simulink model "ECU1119_18b_st"  (R2018b)
settings: Solver=FixedStepDiscrete  StartTime=0.0  StopTime=10.0  RelTol=1e-3
InitFcn:
  | mbd_mpc_consistency_checks(bdroot(gcs));
values from neighbouring files (symbols this model uses):
  ANRtarget = 1.05    [Engine_init.m]
  EGRKi = 0.03    [Engine_init.m]
  EGRKp = 1.2*3    (= 3.6)    [Engine_init.m]
  EGRMax = 1    [Engine_init.m]
  EGRMin = 0    [Engine_init.m]
  EGRTgt = [0.25,0.22,0.20,0.18,0.16,0.12,0.10 ... (first row only)    [Engine_init.m]
  EGRTgt_x = [700,1200,1400,1600,1800,2000,2200]    [Engine_init.m]
  EGRTgt_y = [20,60,100,140,160]    [Engine_init.m]
  EngineSpdTgt = [700:150:2200]    [Engine_init.m]
  EngineSpdTgt_x = [0:10:100]    [Engine_init.m]
  FuelCyleMax = [40,50,60,60,60 ... (first row only)    [Engine_init.m]
  FuelCyleMax_x = [120,180,240,300,360]    [Engine_init.m]
  FuelCyleMax_y = [700,1200,1400,1600,1800,2000,2200]    [Engine_init.m]
  FuelCyleMaxSw = 0    [Engine_init.m]
  FuelCyleMin = 10    [Engine_init.m]
  FuelKd = 0    [Engine_init.m]
  FuelKi = 0.009*5    (= 0.045)    [Engine_init.m]
  FuelKp = 0.03*5    (= 0.15)    [Engine_init.m]
  Regen_Enable_SW = true    [Engine_init.m]
  Soot_Load_Off = 4    [Engine_init.m]
  Soot_Load_On = 18    [Engine_init.m]
  T_regen_max = 680    [Engine_init.m]
  T_regen_min = 550    [Engine_init.m]
undefined symbols (not defined in the file or in its folder): fifo_0_vect, fifo_1_vect, LQFP, pts1_fifo_0_vect, pts1_fifo_1_vect, pts2_fifo_0_vect, pts2_fifo_1_vect, pts3_fifo_0_vect, pts3_fifo_1_vect, pts4_fifo_0_vect, pts4_fifo_1_vect
libraries: mbd_mpc574x_ec_toolbox x111, simulink x12, canmsglib x8
(part 3 of 5)

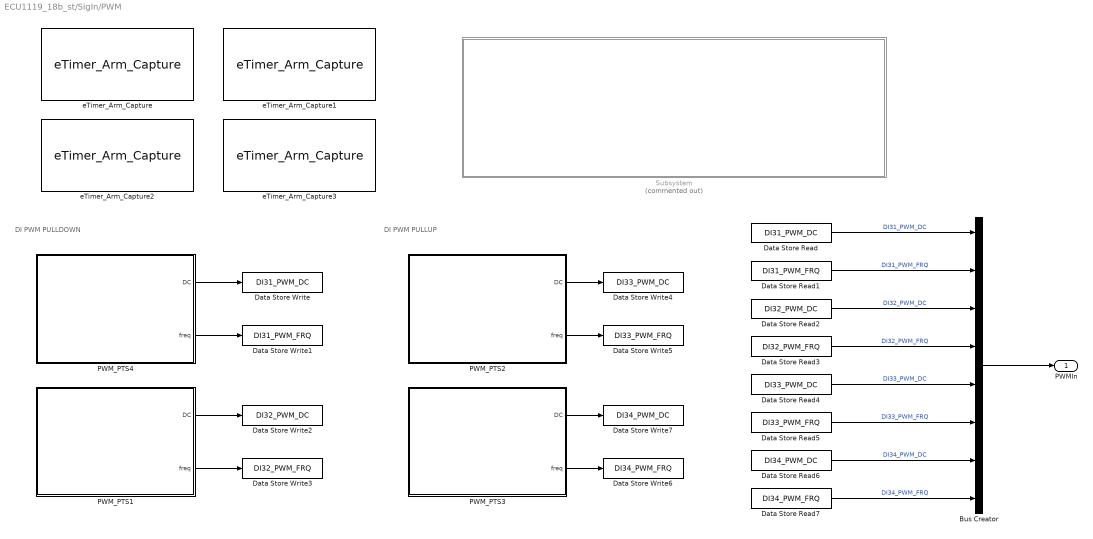
== system ECU1119_18b_st/SigIn/PWM ==
  note: DI PWM PULLDOWN
  note: DI PWM PULLUP
  Bus Creator : BusCreator  Inputs=8
  Data Store Read : DataStoreRead  DataStoreName=DI31_PWM_DC
  Data Store Read1 : DataStoreRead  DataStoreName=DI31_PWM_FRQ
  Data Store Read2 : DataStoreRead  DataStoreName=DI32_PWM_DC
  Data Store Read3 : DataStoreRead  DataStoreName=DI32_PWM_FRQ
  Data Store Read4 : DataStoreRead  DataStoreName=DI33_PWM_DC
  Data Store Read5 : DataStoreRead  DataStoreName=DI33_PWM_FRQ
  Data Store Read6 : DataStoreRead  DataStoreName=DI34_PWM_DC
  Data Store Read7 : DataStoreRead  DataStoreName=DI34_PWM_FRQ
  Data Store Write : DataStoreWrite  DataStoreName=DI31_PWM_DC
  Data Store Write1 : DataStoreWrite  DataStoreName=DI31_PWM_FRQ
  Data Store Write2 : DataStoreWrite  DataStoreName=DI32_PWM_DC
  Data Store Write3 : DataStoreWrite  DataStoreName=DI32_PWM_FRQ
  Data Store Write4 : DataStoreWrite  DataStoreName=DI33_PWM_DC
  Data Store Write5 : DataStoreWrite  DataStoreName=DI33_PWM_FRQ
  Data Store Write6 : DataStoreWrite  DataStoreName=DI34_PWM_FRQ
  Data Store Write7 : DataStoreWrite  DataStoreName=DI34_PWM_DC
  PWM_PTS1 : Subsystem
  PWM_PTS2 : Subsystem
  PWM_PTS3 : Subsystem
  PWM_PTS4 : Subsystem
  Subsystem : Subsystem  Commented=on
  eTimer_Arm_Capture : mbd_mpc574x_ec_toolbox/Motor Control Blocks/eTIMER Blocks/eTimer_Arm_Capture  etimerModule=0  etimerChannel=2  etimerArmAction=Start
      settings: SourceProductName=NXP Model-Based Design Toolbox for MPC57xx MCUs
  eTimer_Arm_Capture1 : mbd_mpc574x_ec_toolbox/Motor Control Blocks/eTIMER Blocks/eTimer_Arm_Capture  etimerModule=1  etimerChannel=2  etimerArmAction=Start
      settings: SourceProductName=NXP Model-Based Design Toolbox for MPC57xx MCUs
  eTimer_Arm_Capture2 : mbd_mpc574x_ec_toolbox/Motor Control Blocks/eTIMER Blocks/eTimer_Arm_Capture  etimerModule=1  etimerChannel=1  etimerArmAction=Start
      settings: SourceProductName=NXP Model-Based Design Toolbox for MPC57xx MCUs
  eTimer_Arm_Capture3 : mbd_mpc574x_ec_toolbox/Motor Control Blocks/eTIMER Blocks/eTimer_Arm_Capture  etimerModule=1  etimerChannel=3  etimerArmAction=Start
      settings: SourceProductName=NXP Model-Based Design Toolbox for MPC57xx MCUs
  PWMIn : Outport
  wires:
  Bus Creator/1 -> PWMIn/1
  Data Store Read7/1 -> Bus Creator/8  "DI34_PWM_FRQ"
  Data Store Read6/1 -> Bus Creator/7  "DI34_PWM_DC"
  Data Store Read5/1 -> Bus Creator/6  "DI33_PWM_FRQ"
  Data Store Read4/1 -> Bus Creator/5  "DI33_PWM_DC"
  Data Store Read3/1 -> Bus Creator/4  "DI32_PWM_FRQ"
  Data Store Read2/1 -> Bus Creator/3  "DI32_PWM_DC"
  Data Store Read1/1 -> Bus Creator/2  "DI31_PWM_FRQ"
  Data Store Read/1 -> Bus Creator/1  "DI31_PWM_DC"
  PWM_PTS4/1(DC) -> Data Store Write/1
  PWM_PTS4/2(freq) -> Data Store Write1/1
  PWM_PTS1/1(DC) -> Data Store Write2/1
  PWM_PTS1/2(freq) -> Data Store Write3/1
  PWM_PTS2/1(DC) -> Data Store Write4/1
  PWM_PTS2/2(freq) -> Data Store Write5/1
  PWM_PTS3/2(freq) -> Data Store Write6/1
  PWM_PTS3/1(DC) -> Data Store Write7/1

== system ECU1119_18b_st/SigOut/VCU_Cmd_Fast ==
  "EngCmd " : Inport
  Trigger : TriggerPort  VariantControl=Variant  PortDimensions=1
  Add : Sum
  Bus Selector : BusSelector  OutputSignals=Data,Length
  Bus Selector1 : BusSelector  OutputSignals=DPF_regen_req,EGROpeningTgt_pct,EngineSpdTgt_rpm,FuelCyleTgt_mg,PostInj_Request
  Constant2 : Constant  OutDataTypeStr=uint8
  Data Store Read : DataStoreRead  DataStoreName=Cnt_FAST_OUT
  Data Store Write : DataStoreWrite  DataStoreName=Cnt_FAST_OUT
  Data Type Conversion{,1..4} (5 alike) : DataTypeConversion  OutDataTypeStr=double
  FCAN_Send_ID_0x18FF0800 : mbd_mpc574x_ec_toolbox/Communication Blocks/CAN Blocks/FCAN_Send  Priority=2  can_instance=2  can_mode=Non-blocking  can_timeout_ms=0  can_mb_idx=6  can_extended_id=off  can_is_remote=off  can_id=107  show_adv_opts=off  can_fd_enable=off  can_enable_brs=off  can_fd_padding=0
      settings: SourceProductName=NXP Model-Based Design Toolbox for MPC57xx MCUs
  VCU_Cmd_Fast : canmsglib/CAN Pack  CANdbFile=D:\VCU\VCU_Tractor_HaerBin\Tractor2\CANtest\ECU_CAN_st.dbc  MsgList=VCU_Cmd_Fast  MsgName=VCU_Cmd_Fast  MsgIDType=Standard (11-bit identifier)  MsgIdentifier=263  MsgLength=8  SignalInfo=DPF_regen_req$56$8$1$2$1$0$1$0$0$1$#EGROpeningTgt_pct$32$16$1$2$1$0$1.000000e-02$0$0$100$#EngSpdTgt_rpm$0$16$1$2$1$0$1.000000e-01$0$0$3000$#FuelCycleTgt_mg$16$16$1$2$1$0$5.000000e-03$0$0$200$#PostInj_Request$48$8$1$2$1$0$1$0$0$1$#  NSignals=5  StartBits=str2num('[int32(56);int32(32);int32(0);int32(16);int32(48)]')  SignalSizes=str2num('[int32(8);int32(16);int32(16);int32(16);int32(8)]')  ByteOrders=str2num('[int32(1);int32(1);int32(1);int32(1);int32(1)]')  DataTypes=str2num('[int32(2);int32(2);int32(2);int32(2);int32(2)]')  MultiplexTypes=str2num('[int32(1);int32(1);int32(1);int32(1);int32(1)]')  MultiplexValues=str2num('[double(0);double(0);double(0);double(0);double(0)]')  Factors=str2num('[double(1);double(1.000000e-02);double(1.000000e-01);double(5.000000e-03);double(1)]')  Offsets=str2num('[double(0);double(0);double(0);double(0);double(0)]')  Minimums=str2num('[double(0);double(0);double(0);double(0);double(0)]')  Maximums=str2num('[double(1);double(100);double(3000);double(200);double(1)]')  Remote=off  ApplyMinMax=off  BusOutput=on
      settings: SourceProductName=Simulink Real-Time  SourceProductBaseCode=XP  DataFormat=CANdb specified signals
  wires:
  VCU_Cmd_Fast/1 -> Bus Selector/1
  Bus Selector/2 -> FCAN_Send_ID_0x18FF0800/2  "<Length>"
  Bus Selector/1 -> FCAN_Send_ID_0x18FF0800/1  "<Data>"
  Add/1 -> Data Store Write/1
  Data Store Read/1 -> Add/1
  Constant2/1 -> Add/2
  "EngCmd "/1 -> Bus Selector1/1
  Data Type Conversion/1 -> VCU_Cmd_Fast/1
  Data Type Conversion4/1 -> VCU_Cmd_Fast/5
  Data Type Conversion3/1 -> VCU_Cmd_Fast/4
  Data Type Conversion2/1 -> VCU_Cmd_Fast/3
  Data Type Conversion1/1 -> VCU_Cmd_Fast/2
  Bus Selector1/5 -> Data Type Conversion4/1  "<PostInj_Request>"
  Bus Selector1/4 -> Data Type Conversion3/1  "<FuelCyleTgt_mg>"
  Bus Selector1/3 -> Data Type Conversion2/1  "<EngineSpdTgt_rpm>"
  Bus Selector1/2 -> Data Type Conversion1/1  "<EGROpeningTgt_pct>"
  Bus Selector1/1 -> Data Type Conversion/1  "<DPF_regen_req>"

== system ECU1119_18b_st/SigOut/VCU_Cmd_Slow ==
  "EngCmd " : Inport
  Trigger : TriggerPort  VariantControl=Variant  PortDimensions=1
  Add : Sum
  Bus Selector : BusSelector  OutputSignals=Data,Length
  Bus Selector1 : BusSelector  OutputSignals=mUREA_target
  Constant : Constant  Value=0  OutDataTypeStr=single
  Constant2 : Constant  OutDataTypeStr=uint8
  Data Store Read : DataStoreRead  DataStoreName=Cnt_SLOW_OUT
  Data Store Write : DataStoreWrite  DataStoreName=Cnt_SLOW_OUT
  Data Type Conversion : DataTypeConversion  OutDataTypeStr=double
  Data Type Conversion1 : DataTypeConversion  OutDataTypeStr=double
  FCAN_Send_ID_0x18FF0900 : mbd_mpc574x_ec_toolbox/Communication Blocks/CAN Blocks/FCAN_Send  Priority=2  can_instance=2  can_mode=Non-blocking  can_timeout_ms=0  can_mb_idx=7  can_extended_id=off  can_is_remote=off  can_id=108  show_adv_opts=off  can_fd_enable=off  can_enable_brs=off  can_fd_padding=0
      settings: SourceProductName=NXP Model-Based Design Toolbox for MPC57xx MCUs
  VCU_Cmd_Slow : canmsglib/CAN Pack  CANdbFile=D:\VCU\VCU_Tractor_HaerBin\Tractor2\CANtest\ECU_CAN_st.dbc  MsgList=VCU_Cmd_Slow  MsgName=VCU_Cmd_Slow  MsgIDType=Standard (11-bit identifier)  MsgIdentifier=264  MsgLength=8  SignalInfo=Reserved_0900$0$32$1$3$1$0$1$0$-3.400000e+38$3.400000e+38$#mUREA_target_gph$32$32$1$3$1$0$1.000000e-01$0$-3.400000e+37$3.400000e+37$#  NSignals=2  StartBits=str2num('[int32(0);int32(32)]')  SignalSizes=str2num('[int32(32);int32(32)]')  ByteOrders=str2num('[int32(1);int32(1)]')  DataTypes=str2num('[int32(3);int32(3)]')  MultiplexTypes=str2num('[int32(1);int32(1)]')  MultiplexValues=str2num('[double(0);double(0)]')  Factors=str2num('[double(1);double(1.000000e-01)]')  Offsets=str2num('[double(0);double(0)]')  Minimums=str2num('[double(-3.400000e+38);double(-3.400000e+37)]')  Maximums=str2num('[double(3.400000e+38);double(3.400000e+37)]')  Remote=off  ApplyMinMax=off  BusOutput=on
      settings: SourceProductName=Simulink Real-Time  SourceProductBaseCode=XP  DataFormat=CANdb specified signals
  wires:
  Bus Selector1/1 -> Data Type Conversion/1  "<mUREA_target>"
  "EngCmd "/1 -> Bus Selector1/1
  Constant2/1 -> Add/2
  Data Store Read/1 -> Add/1
  Add/1 -> Data Store Write/1
  Bus Selector/1 -> FCAN_Send_ID_0x18FF0900/1  "<Data>"
  Bus Selector/2 -> FCAN_Send_ID_0x18FF0900/2  "<Length>"
  VCU_Cmd_Slow/1 -> Bus Selector/1
  Data Type Conversion/1 -> VCU_Cmd_Slow/2
  Data Type Conversion1/1 -> VCU_Cmd_Slow/1
  Constant/1 -> Data Type Conversion1/1

== system ECU1119_18b_st/ECU/ECU/ANR ==
  note: 当前框图逻辑没有错误，能跑；但属于开环前馈方案，不是工程上的储氨闭环 SCR 控制。
  note: 工程上是 SCR 温度的二维查表 MAP ：ExhTemp_DPF_out → ANR 目标（一般 0.8~1.05），低温段 ANR 压低，避免 NH3 逃逸；你现在固定 1，简化仿真可以跑，但如果要看氨逃逸指标，必须改成查表。
  note: 控制需求的氨供给流量，
      | 由 ANR×NOx 决定
  ExhTemp_DPF_out : Inport
  mNOx_SCR_kg/h : Inport  Port=2
  ANRtarget : Constant  Value=ANRtarget
  Divide : Product  Inputs=*/
  Product : Product
  Relational Operator : RelationalOperator  Operator=<=  OutDataTypeStr=boolean  RndMeth=Simplest
  Switch : Switch  Criteria=u2 > Threshold
  zero2 : Constant  Value=0
  低温 : Constant  Value=200
  尿素浓度 : Constant  Value=0.325
  mUREA_target : Outport  VectorParamsAs1DForOutWhenUnconnected=on
  wires:
  Relational Operator/1 -> Switch/2
  低温/1 -> Relational Operator/2
  ANRtarget/1 -> Product/1
  尿素浓度/1 -> Divide/2
  ExhTemp_DPF_out/1 -> Relational Operator/1
  Divide/1 -> Switch/3
  zero2/1 -> Switch/1
  Product/1 -> Divide/1  "mNH3_target"
  mNOx_SCR_kg/h/1 -> Product/2
  Switch/1 -> mUREA_target/1  "mUREA_target"

== system ECU1119_18b_st/ECU/ECU/DPF_REGEN ==
  note: 0 待机，1 条件满足等待，2 再生中，3 再生退出 / 故障
  ExhTemp_DOC_out : Inport
  ExhTemp_DPF_out : Inport  Port=2
  DPF_SootLoad : Inport  Port=3
  ExhMassFlow : Inport  Port=4
  DPF_DP : Inport  Port=5
  EngineSpd_rpm : Inport  Port=6
  Chart : Stateflow chart  TreatAsAtomicUnit=on
  Terminator{,1..3} (4 alike) : Terminator
  DPF_regen_req : Outport  VectorParamsAs1DForOutWhenUnconnected=on
  PostInj_Request : Outport  Port=2  VectorParamsAs1DForOutWhenUnconnected=on
  Regen_State : Outport  Port=3  VectorParamsAs1DForOutWhenUnconnected=on
  wires:
  DPF_SootLoad/1 -> Chart/1(DPF_SootLoad)
  ExhTemp_DOC_out/1 -> Chart/2(ExhTemp_DPF_in_c)
  ExhTemp_DPF_out/1 -> Terminator/1
  ExhMassFlow/1 -> Terminator1/1
  EngineSpd_rpm/1 -> Terminator3/1
  DPF_DP/1 -> Terminator2/1
  Chart/1(Regen_Request) -> DPF_regen_req/1
  Chart/3(PostInj_Request) -> PostInj_Request/1
  Chart/2(Regen_State) -> Regen_State/1

== system ECU1119_18b_st/ECU/ECU/EGRCtrl ==
  note: - 当 **实际 EGR 率 < 目标 EGR 率**（EGR 不够）：
      | 偏差 > 0- PID 输入正偏差 → PID 输出变大 → EGR 阀开度变大
  note: EGR 率 = 回流废气质量 / 总进气质量，范围 0~0.3，标注正确。
  note: PID 输出 0~1，乘以 100 转为百分比开度 EGROpeningTgt_pct ；上下限 EGRMax/EGRMin 限幅；
  note: 实际 EGRRatio
  note: 目标 EGR 率
  note: EGR 率：回流废气质量 / 总进气质量
      | 一般 0~30% 左右
  EngineSpd_rpm : Inport
  FuleCycle_mg : Inport  Port=2
  EGRRatio : Inport  Port=3
  Add : Sum  Inputs=+-
  Constant : Constant  Value=EGRKp
  Constant1 : Constant  Value=EGRKi
  Constant2 : Constant  Value=0.01
  Constant3 : Constant  Value=100
  Constant4 : Constant  Value=EGRMin
  Constant5 : Constant  Value=EGRMax
  EGRTgt : Lookup_n-D  BreakpointsForDimension1=EGRTgt_x  BreakpointsForDimension2=EGRTgt_y  Table=EGRTgt  ExtrapMethod=Clip  InternalRulePriority=Speed  RndMeth=Simplest  InputSameDT=on
  Gain : Gain  Gain=100
  Gain1 : Gain  Gain=30
  Gain2 : Gain  Gain=0.5
  Mux : Mux  Inputs=2
  PID Controller : simulink/Continuous/PID Controller  Controller=PID  Form=Parallel  TimeDomain=Discrete-time  SampleTime=-1  IntegratorMethod=Forward Euler  FilterMethod=Forward Euler  ControllerParametersSource=external  P=1  I=1  D=0  UseFilter=on  N=100  TunerSelectOption=Transfer Function Based (PID Tuner App)  InitialConditionSource=internal  InitialConditionForIntegrator=0  InitialConditionForFilter=0  DifferentiatorICPrevScaledInput=0  ExternalReset=none  TrackingMode=off  Kt=1  LimitOutput=on  UpperSaturationLimit=1  LowerSaturationLimit=0  LinearizeAsGain=on  AntiWindupMode=back-calculation  Kb=1  POutMin=[]  POutMax=[]  IOutMin=[]  IOutMax=[]  DOutMin=[]  DOutMax=[]  NOutMin=[]  NOutMax=[]  SumOutMin=[]  SumOutMax=[]  SaturationOutMin=[]  SaturationOutMax=[]  PParamMin=[]  PParamMax=[]  IParamMin=[]  IParamMax=[]  DParamMin=[]  DParamMax=[]  NParamMin=[]  NParamMax=[]  KbParamMin=[]  KbParamMax=[]  KtParamMin=[]  KtParamMax=[]  KbOutMin=[]  KbOutMax=[]  KtOutMin=[]  KtOutMax=[]  IntegratorOutMin=[]  IntegratorOutMax=[]  FilterOutMin=[]  FilterOutMax=[]  SumI1OutMin=[]  SumI1OutMax=[]  SumI2OutMin=[]  SumI2OutMax=[]  SumI3OutMin=[]  SumI3OutMax=[]  SumI4OutMin=[]  SumI4OutMax=[]  SumDOutMin=[]  SumDOutMax=[]  DifferentiatorOutMin=[]  DifferentiatorOutMax=[]  FilterDiffOutCoefMin=[]  FilterDiffOutCoefMax=[]  ReciprocalOutMin=[]  ReciprocalOutMax=[]  SumDenOutMin=[]  SumDenOutMax=[]  SumNumOutMin=[]  SumNumOutMax=[]  DivideOutMin=[]  DivideOutMax=[]  IntegratorContinuousStateAttributes=''  IntegratorStateMustResolveToSignalObject=off  IntegratorRTWStateStorageClass=Auto  FilterContinuousStateAttributes=''  FilterStateMustResolveToSignalObject=off  FilterRTWStateStorageClass=Auto  ParallelPVariant=ExternalParameters  IdealPVariant=Disabled  IVariant=ExternalParameters  DVariant=ExternalParameters  IntegratorVariant=Discrete  SatVariant=Enabled  AWVariant=BackCalculation  PCopyVariant=Disabled  TRVariant=Disabled  FdbkBlocksVariant=Forward  IdealPFdbkVariant=Disabled  SatFdbkVariant=Disabled  DerivativeFilterVariant=ForwardEulerFilter  NVariant=ExternalParameters  NCopyVariant=Disabled  FilterICVariant=InternalICsFilter  IntegratorICVariant=InternalICs  ExternalResetVariant=Disabled  TRSumVariant=Passthrough  SumFdbkVariant=Disabled  SumVariant=Sum_PID
  Scope : Scope  NumInputPorts=4
  Terminator : Terminator
  Terminator1 : Terminator
  EGROpeningTgt_pct : Outport  VectorParamsAs1DForOutWhenUnconnected=on
  wires:
  Add/1 -> PID Controller/1  "EGRErr"
  Constant2/1 -> PID Controller/4
  Constant4/1 -> Terminator1/1
  Constant3/1 -> PID Controller/5
  EGRRatio/1 -> Mux/2, Add/2  "EGRRatio"
  Constant/1 -> Gain2/1
  EGRTgt/1 -> Mux/1, Add/1  "EGRTgt"
  Constant1/1 -> Gain1/1
  PID Controller/1 -> Gain/1
  Constant5/1 -> Terminator/1
  EngineSpd_rpm/1 -> Scope/1, EGRTgt/1  "EngineSpd_rpm"
  FuleCycle_mg/1 -> Scope/2, EGRTgt/2  "FuleCycle_mg"
  Gain/1 -> Scope/4, EGROpeningTgt_pct/1  "EGROpeningTgt_pct"
  Mux/1 -> Scope/3
  Gain1/1 -> PID Controller/3
  Gain2/1 -> PID Controller/2

== system ECU1119_18b_st/ECU/ECU/SpdCtrl ==
  note: 允许最大喷油量
  note: 冒烟限制 MAP
  ThrottleCmd_pct : Inport
  EngineSpd_rpm : Inport  Port=2
  RailPrs_kpa : Inport  Port=3
  IntakeMass : Inport  Port=4
  Add : Sum  Inputs=+-
  Constant : Constant  Value=FuelKp
  Constant1 : Constant  Value=FuelKi
  Constant2 : Constant  Value=FuelKd
  Constant3 : Constant  Value=100
  Constant4 : Constant  Value=FuelCyleMin
  Constant5 : Constant  Value=160
  Constant6 : Constant  Value=FuelCyleMaxSw
  EngineSpdTgt : Lookup_n-D  NumberOfTableDimensions=1  BreakpointsForDimension1=EngineSpdTgt_x  Table=EngineSpdTgt  ExtrapMethod=Clip  InternalRulePriority=Speed  RndMeth=Simplest  InputSameDT=on
  FuelCyleMax : Lookup_n-D  BreakpointsForDimension1=FuelCyleMax_x  BreakpointsForDimension2=FuelCyleMax_y  Table=FuelCyleMax  ExtrapMethod=Clip  InternalRulePriority=Speed  RndMeth=Simplest  InputSameDT=on
  Mux : Mux  Inputs=2
  PID Controller : simulink/Continuous/PID Controller  Controller=PID  Form=Parallel  TimeDomain=Discrete-time  SampleTime=-1  IntegratorMethod=Forward Euler  FilterMethod=Forward Euler  ControllerParametersSource=external  P=1  I=1  D=0  UseFilter=on  N=100  TunerSelectOption=Transfer Function Based (PID Tuner App)  InitialConditionSource=internal  InitialConditionForIntegrator=0  InitialConditionForFilter=0  DifferentiatorICPrevScaledInput=0  ExternalReset=none  TrackingMode=off  Kt=1  LimitOutput=on  UpperSaturationLimit=inf  LowerSaturationLimit=-inf  LinearizeAsGain=on  AntiWindupMode=back-calculation  Kb=1  POutMin=[]  POutMax=[]  IOutMin=[]  IOutMax=[]  DOutMin=[]  DOutMax=[]  NOutMin=[]  NOutMax=[]  SumOutMin=[]  SumOutMax=[]  SaturationOutMin=[]  SaturationOutMax=[]  PParamMin=[]  PParamMax=[]  IParamMin=[]  IParamMax=[]  DParamMin=[]  DParamMax=[]  NParamMin=[]  NParamMax=[]  KbParamMin=[]  KbParamMax=[]  KtParamMin=[]  KtParamMax=[]  KbOutMin=[]  KbOutMax=[]  KtOutMin=[]  KtOutMax=[]  IntegratorOutMin=[]  IntegratorOutMax=[]  FilterOutMin=[]  FilterOutMax=[]  SumI1OutMin=[]  SumI1OutMax=[]  SumI2OutMin=[]  SumI2OutMax=[]  SumI3OutMin=[]  SumI3OutMax=[]  SumI4OutMin=[]  SumI4OutMax=[]  SumDOutMin=[]  SumDOutMax=[]  DifferentiatorOutMin=[]  DifferentiatorOutMax=[]  FilterDiffOutCoefMin=[]  FilterDiffOutCoefMax=[]  ReciprocalOutMin=[]  ReciprocalOutMax=[]  SumDenOutMin=[]  SumDenOutMax=[]  SumNumOutMin=[]  SumNumOutMax=[]  DivideOutMin=[]  DivideOutMax=[]  IntegratorContinuousStateAttributes=''  IntegratorStateMustResolveToSignalObject=off  IntegratorRTWStateStorageClass=Auto  FilterContinuousStateAttributes=''  FilterStateMustResolveToSignalObject=off  FilterRTWStateStorageClass=Auto  ParallelPVariant=ExternalParameters  IdealPVariant=Disabled  IVariant=ExternalParameters  DVariant=ExternalParameters  IntegratorVariant=Discrete  SatVariant=Enabled  AWVariant=BackCalculation  PCopyVariant=Disabled  TRVariant=Disabled  FdbkBlocksVariant=Forward  IdealPFdbkVariant=Disabled  SatFdbkVariant=Disabled  DerivativeFilterVariant=ForwardEulerFilter  NVariant=ExternalParameters  NCopyVariant=Disabled  FilterICVariant=InternalICsFilter  IntegratorICVariant=InternalICs  ExternalResetVariant=Disabled  TRSumVariant=Passthrough  SumFdbkVariant=Disabled  SumVariant=Sum_PID
  Saturation Dynamic : simulink/Discontinuities/Saturation Dynamic  OutMin=[]  OutMax=[]  OutDataTypeStr=Inherit: Same as second input  OutDataType=fixdt(1, 16)  OutScaling=2^-10  DoSatur=off
  Scope : Scope  NumInputPorts=3
  Switch : Switch  Criteria=u2 > Threshold
  Terminator : Terminator
  FuelCycle_mg : Outport  VectorParamsAs1DForOutWhenUnconnected=on
  EngineSpdTgt_rpm : Outport  Port=2  VectorParamsAs1DForOutWhenUnconnected=on
  wires:
  EngineSpd_rpm/1 -> Mux/2, Add/2, FuelCyleMax/2
  Add/1 -> PID Controller/1
  PID Controller/1 -> Saturation Dynamic/2, Scope/3
  Constant/1 -> PID Controller/2
  Constant1/1 -> PID Controller/3
  Constant3/1 -> PID Controller/5
  Constant2/1 -> PID Controller/4
  Constant4/1 -> Saturation Dynamic/3
  IntakeMass/1 -> FuelCyleMax/1
  RailPrs_kpa/1 -> Terminator/1
  Switch/1 -> Saturation Dynamic/1
  FuelCyleMax/1 -> Switch/1
  Constant5/1 -> Switch/3
  Constant6/1 -> Switch/2
  ThrottleCmd_pct/1 -> EngineSpdTgt/1, Scope/1
  EngineSpdTgt/1 -> EngineSpdTgt_rpm/1, Mux/1, Add/1
  Mux/1 -> Scope/2
  Saturation Dynamic/1 -> FuelCycle_mg/1

== system ECU1119_18b_st/GPIO /ETC/Subsystem ==
  COMPLD1 : Inport
  COMPLD2 : Inport  Port=2
  Constant4 : Constant  Value=0  OutDataTypeStr=Inherit: Inherit via back propagation
  Data Type Conversion : DataTypeConversion
  Data Type Conversion1 : DataTypeConversion
  Data Type Conversion2 : DataTypeConversion
  eTimer_Preload2 : mbd_mpc574x_ec_toolbox/Motor Control Blocks/eTIMER Blocks/eTimer_Preload  etimerModule=0  etimerChannel=3
      settings: SourceProductName=NXP Model-Based Design Toolbox for MPC57xx MCUs
  eTimer_Start_Stop_Timer1 : mbd_mpc574x_ec_toolbox/Motor Control Blocks/eTIMER Blocks/eTimer_Start_Stop_Timer  etimerModule=0  etimerChannel=3  etimerAction=Start
      settings: SourceProductName=NXP Model-Based Design Toolbox for MPC57xx MCUs
  wires:
  Constant4/1 -> Data Type Conversion/1
  COMPLD2/1 -> Data Type Conversion2/1
  COMPLD1/1 -> Data Type Conversion1/1
  Data Type Conversion/1 -> eTimer_Preload2/1
  Data Type Conversion1/1 -> eTimer_Preload2/2
  Data Type Conversion2/1 -> eTimer_Preload2/3

== system ECU1119_18b_st/GPIO /ETC/Subsystem1 ==
  COMPLD1 : Inport
  COMPLD2 : Inport  Port=2
  Constant4 : Constant  Value=0  OutDataTypeStr=Inherit: Inherit via back propagation
  Data Type Conversion : DataTypeConversion
  Data Type Conversion1 : DataTypeConversion
  Data Type Conversion2 : DataTypeConversion
  eTimer_Preload2 : mbd_mpc574x_ec_toolbox/Motor Control Blocks/eTIMER Blocks/eTimer_Preload  etimerModule=2  etimerChannel=2
      settings: SourceProductName=NXP Model-Based Design Toolbox for MPC57xx MCUs
  eTimer_Start_Stop_Timer1 : mbd_mpc574x_ec_toolbox/Motor Control Blocks/eTIMER Blocks/eTimer_Start_Stop_Timer  etimerModule=2  etimerChannel=2  etimerAction=Start
      settings: SourceProductName=NXP Model-Based Design Toolbox for MPC57xx MCUs
  wires:
  COMPLD1/1 -> Data Type Conversion1/1
  COMPLD2/1 -> Data Type Conversion2/1
  Constant4/1 -> Data Type Conversion/1
  Data Type Conversion/1 -> eTimer_Preload2/1
  Data Type Conversion1/1 -> eTimer_Preload2/2
  Data Type Conversion2/1 -> eTimer_Preload2/3

== system ECU1119_18b_st/GPIO /ETC/Subsystem2 ==
  COMPLD1 : Inport
  COMPLD2 : Inport  Port=2
  Constant4 : Constant  Value=0  OutDataTypeStr=Inherit: Inherit via back propagation
  Data Type Conversion : DataTypeConversion
  Data Type Conversion1 : DataTypeConversion
  Data Type Conversion2 : DataTypeConversion
  eTimer_Preload2 : mbd_mpc574x_ec_toolbox/Motor Control Blocks/eTIMER Blocks/eTimer_Preload  etimerModule=0  etimerChannel=5
      settings: SourceProductName=NXP Model-Based Design Toolbox for MPC57xx MCUs
  eTimer_Start_Stop_Timer1 : mbd_mpc574x_ec_toolbox/Motor Control Blocks/eTIMER Blocks/eTimer_Start_Stop_Timer  etimerModule=0  etimerChannel=5  etimerAction=Start
      settings: SourceProductName=NXP Model-Based Design Toolbox for MPC57xx MCUs
  wires:
  Constant4/1 -> Data Type Conversion/1
  COMPLD2/1 -> Data Type Conversion2/1
  COMPLD1/1 -> Data Type Conversion1/1
  Data Type Conversion/1 -> eTimer_Preload2/1
  Data Type Conversion1/1 -> eTimer_Preload2/2
  Data Type Conversion2/1 -> eTimer_Preload2/3

== system ECU1119_18b_st/GPIO /ETC/Subsystem3 ==
  COMPLD1 : Inport
  COMPLD2 : Inport  Port=2
  Constant4 : Constant  Value=0  OutDataTypeStr=Inherit: Inherit via back propagation
  Data Type Conversion : DataTypeConversion
  Data Type Conversion1 : DataTypeConversion
  Data Type Conversion2 : DataTypeConversion
  eTimer_Preload2 : mbd_mpc574x_ec_toolbox/Motor Control Blocks/eTIMER Blocks/eTimer_Preload  etimerModule=1  etimerChannel=4
      settings: SourceProductName=NXP Model-Based Design Toolbox for MPC57xx MCUs
  eTimer_Start_Stop_Timer1 : mbd_mpc574x_ec_toolbox/Motor Control Blocks/eTIMER Blocks/eTimer_Start_Stop_Timer  etimerModule=1  etimerChannel=4  etimerAction=Start
      settings: SourceProductName=NXP Model-Based Design Toolbox for MPC57xx MCUs
  wires:
  Data Type Conversion2/1 -> eTimer_Preload2/3
  Data Type Conversion1/1 -> eTimer_Preload2/2
  Data Type Conversion/1 -> eTimer_Preload2/1
  COMPLD1/1 -> Data Type Conversion1/1
  COMPLD2/1 -> Data Type Conversion2/1
  Constant4/1 -> Data Type Conversion/1

== system ECU1119_18b_st/GPIO /ETC/Subsystem4 ==
  COMPLD1 : Inport
  COMPLD2 : Inport  Port=2
  Constant4 : Constant  Value=0  OutDataTypeStr=Inherit: Inherit via back propagation
  Data Type Conversion : DataTypeConversion
  Data Type Conversion1 : DataTypeConversion
  Data Type Conversion2 : DataTypeConversion
  eTimer_Preload2 : mbd_mpc574x_ec_toolbox/Motor Control Blocks/eTIMER Blocks/eTimer_Preload  etimerModule=1  etimerChannel=5
      settings: SourceProductName=NXP Model-Based Design Toolbox for MPC57xx MCUs
  eTimer_Start_Stop_Timer1 : mbd_mpc574x_ec_toolbox/Motor Control Blocks/eTIMER Blocks/eTimer_Start_Stop_Timer  etimerModule=1  etimerChannel=5  etimerAction=Start
      settings: SourceProductName=NXP Model-Based Design Toolbox for MPC57xx MCUs
  wires:
  Data Type Conversion2/1 -> eTimer_Preload2/3
  Data Type Conversion1/1 -> eTimer_Preload2/2
  Data Type Conversion/1 -> eTimer_Preload2/1
  Constant4/1 -> Data Type Conversion/1
  COMPLD2/1 -> Data Type Conversion2/1
  COMPLD1/1 -> Data Type Conversion1/1

== system ECU1119_18b_st/GPIO /ETC/Subsystem5 ==
  COMPLD1 : Inport
  COMPLD2 : Inport  Port=2
  Constant4 : Constant  Value=0  OutDataTypeStr=Inherit: Inherit via back propagation
  Data Type Conversion : DataTypeConversion
  Data Type Conversion1 : DataTypeConversion
  Data Type Conversion2 : DataTypeConversion
  eTimer_Preload2 : mbd_mpc574x_ec_toolbox/Motor Control Blocks/eTIMER Blocks/eTimer_Preload  etimerModule=1  etimerChannel=0
      settings: SourceProductName=NXP Model-Based Design Toolbox for MPC57xx MCUs
  eTimer_Start_Stop_Timer1 : mbd_mpc574x_ec_toolbox/Motor Control Blocks/eTIMER Blocks/eTimer_Start_Stop_Timer  etimerModule=1  etimerChannel=0  etimerAction=Start
      settings: SourceProductName=NXP Model-Based Design Toolbox for MPC57xx MCUs
  wires:
  Data Type Conversion2/1 -> eTimer_Preload2/3
  Data Type Conversion1/1 -> eTimer_Preload2/2
  Data Type Conversion/1 -> eTimer_Preload2/1
  COMPLD1/1 -> Data Type Conversion1/1
  COMPLD2/1 -> Data Type Conversion2/1
  Constant4/1 -> Data Type Conversion/1

== system ECU1119_18b_st/GPIO /PWM_OUT/PWM Configuration and Frequency Update ==
  In1 : Inport
  In2 : Inport  Port=2
  FlexPWM_Config : mbd_mpc574x_ec_toolbox/Motor Control Blocks/FlexPWM Blocks/FlexPWM_Config  Priority=1  pwmModule=0  pwmSubmodule=3  pwmMode=Edge aligned PWM  pwmPair=Independent  pwmCompSource=PWM23  pwmCounterInit=Local sync (PWMX)  pwmClockSource=Peripheral clock  pwmUnits=Hz  pwmFrequency=10000  pwmPeriod=8000  pwmPrescaler=Divide by 1  pwmDtUnits=Nanoseconds  pwmDtNs=50  pwmDtTicks=4  pwmReloadLogic=Full Cycle  pwmReloadFrequency=Every 1 PWM opportunity  pwmTriggeringSignal=Local force signal  pwmDutyCycleOutSim=off  pwmStartAfterInit=on  pwmShowAdvOpts=off  pwmPinA=PTA2: [PWM0_A3 | FlexPWM_0 Channel A Input/Output 3]  pwmPinB=None  pwmPolarityA=off  pwmPolarityB=off  pwmAInitialVal=0.25  pwmBInitialVal=0.25  pwmAShift=0  pwmBShift=0  trgReloadISR=off  trgVal0=off  trgVal1=off  trgVal2=off  trgVal3=off  trgVal4=off  trgVal5=off  trgReloadErrorISR=off  pwmPinFault=None  PwmFaultEnISR=off  pwmFaultEnA=off  pwmFaultEnB=off
      settings: SourceProductName=NXP Model-Based Design Toolbox for MPC57xx MCUs
  FlexPWM_Frequency_Update : mbd_mpc574x_ec_toolbox/Motor Control Blocks/FlexPWM Blocks/FlexPWM_Frequency_Update  Priority=1  pwmModule=0  pwmSubmodule0=off  pwmSubmodule1=off  pwmSubmodule2=off  pwmSubmodule3=on  pwmUnits=Hz
      settings: SourceProductName=NXP Model-Based Design Toolbox for MPC57xx MCUs
  wires:
  In1/1 -> FlexPWM_Frequency_Update/1
  In2/1 -> FlexPWM_Config/1

== system ECU1119_18b_st/GPIO /PWM_OUT/PWM Configuration and Frequency Update1 ==
  PWM A : Inport
  Fre A : Inport  Port=2
  PWM B : Inport  Port=3
  Fre B : Inport  Port=4
  Constant2 : Constant  Commented=on  Value=200
  Data Type Conversion : DataTypeConversion
  Data Type Conversion1 : DataTypeConversion
  Data Type Conversion2 : DataTypeConversion  Commented=on
  FlexPWM_Config : mbd_mpc574x_ec_toolbox/Motor Control Blocks/FlexPWM Blocks/FlexPWM_Config  Priority=1  pwmModule=0  pwmSubmodule=3  pwmMode=Center aligned PWM  pwmPair=Independent  pwmCompSource=PWM23  pwmCounterInit=Local sync (PWMX)  pwmClockSource=Peripheral clock  pwmUnits=Hz  pwmFrequency=200  pwmPeriod=25000  pwmPrescaler=Divide by 16  pwmDtUnits=Nanoseconds  pwmDtNs=50  pwmDtTicks=4  pwmReloadLogic=Full Cycle  pwmReloadFrequency=Every 1 PWM opportunity  pwmTriggeringSignal=Local force signal  pwmDutyCycleOutSim=off  pwmStartAfterInit=on  pwmShowAdvOpts=off  pwmPinA=PTD3: [PWM0_A3 | FlexPWM_0 Channel A Input/Output 3]  pwmPinB=PTD4: [PWM0_B3 | FlexPWM_0 Channel B Input/Output 3]  pwmPolarityA=off  pwmPolarityB=off  pwmAInitialVal=0.5  pwmBInitialVal=0.25  pwmAShift=0  pwmBShift=0  trgReloadISR=off  trgVal0=off  trgVal1=off  trgVal2=off  trgVal3=off  trgVal4=off  trgVal5=off  trgReloadErrorISR=off  pwmPinFault=None  PwmFaultEnISR=off  pwmFaultEnA=off  pwmFaultEnB=off
      settings: SourceProductName=NXP Model-Based Design Toolbox for MPC57xx MCUs
  FlexPWM_Frequency_Update : mbd_mpc574x_ec_toolbox/Motor Control Blocks/FlexPWM Blocks/FlexPWM_Frequency_Update  Priority=1  Commented=on  pwmModule=0  pwmSubmodule0=off  pwmSubmodule1=off  pwmSubmodule2=off  pwmSubmodule3=on  pwmUnits=Hz
      settings: SourceProductName=NXP Model-Based Design Toolbox for MPC57xx MCUs
  Terminator : Terminator
  Terminator1 : Terminator
  wires:
  Fre B/1 -> Terminator/1
  PWM A/1 -> Data Type Conversion/1
  Data Type Conversion/1 -> FlexPWM_Config/1
  PWM B/1 -> Data Type Conversion1/1
  Data Type Conversion1/1 -> FlexPWM_Config/2
  Fre A/1 -> Terminator1/1
  Constant2/1 -> Data Type Conversion2/1
  Data Type Conversion2/1 -> FlexPWM_Frequency_Update/1

== system ECU1119_18b_st/GPIO /PWM_OUT/PWM Configuration and Frequency Update4 ==
  PWM A : Inport
  Fre : Inport  Port=2
  Add : Sum  Inputs=+-
  Constant : Constant
  Constant1 : Constant  Commented=on  Value=200
  Data Type Conversion : DataTypeConversion
  Data Type Conversion1 : DataTypeConversion  Commented=on
  FlexPWM_Config : mbd_mpc574x_ec_toolbox/Motor Control Blocks/FlexPWM Blocks/FlexPWM_Config  Priority=1  pwmModule=0  pwmSubmodule=1  pwmMode=Center aligned PWM  pwmPair=Independent  pwmCompSource=PWM23  pwmCounterInit=Local sync (PWMX)  pwmClockSource=Peripheral clock  pwmUnits=Hz  pwmFrequency=200  pwmPeriod=25000  pwmPrescaler=Divide by 16  pwmDtUnits=Nanoseconds  pwmDtNs=50  pwmDtTicks=4  pwmReloadLogic=Full Cycle  pwmReloadFrequency=Every 1 PWM opportunity  pwmTriggeringSignal=Local force signal  pwmDutyCycleOutSim=off  pwmStartAfterInit=on  pwmShowAdvOpts=off  pwmPinA=PTC7: [PWM0_A1 | FlexPWM_0 Channel A Input/Output 1]  pwmPinB=None  pwmPolarityA=off  pwmPolarityB=off  pwmAInitialVal=0.25  pwmBInitialVal=0.25  pwmAShift=0  pwmBShift=0  trgReloadISR=off  trgVal0=off  trgVal1=off  trgVal2=off  trgVal3=off  trgVal4=off  trgVal5=off  trgReloadErrorISR=off  pwmPinFault=None  PwmFaultEnISR=off  pwmFaultEnA=off  pwmFaultEnB=off
      settings: SourceProductName=NXP Model-Based Design Toolbox for MPC57xx MCUs
  FlexPWM_Frequency_Update : mbd_mpc574x_ec_toolbox/Motor Control Blocks/FlexPWM Blocks/FlexPWM_Frequency_Update  Priority=1  Commented=on  pwmModule=0  pwmSubmodule0=off  pwmSubmodule1=on  pwmSubmodule2=off  pwmSubmodule3=off  pwmUnits=Hz
      settings: SourceProductName=NXP Model-Based Design Toolbox for MPC57xx MCUs
  Terminator : Terminator
  wires:
  PWM A/1 -> Add/2
  Add/1 -> Data Type Conversion/1
  Constant/1 -> Add/1
  Data Type Conversion/1 -> FlexPWM_Config/1
  Fre/1 -> Terminator/1
  Constant1/1 -> Data Type Conversion1/1
  Data Type Conversion1/1 -> FlexPWM_Frequency_Update/1

== system ECU1119_18b_st/GPIO /SPI0: LS09_14_15_16_1_2_11_4/LS_CTRL ==
  Enable : EnablePort
  Data Type Conversion3 : DataTypeConversion
  Data Type Conversion4 : DataTypeConversion
  Demux1 : Demux  Outputs=2
  If Action Subsystem1 : Subsystem  TreatAsAtomicUnit=on
  SPI_Master_Transfer_To1 : mbd_mpc574x_ec_toolbox/Communication Blocks/SPI Blocks/SPI_Master_Transfer  Priority=2  InstanceNumber=0  xfermode=Non blocking  timeout=50  spi_upd=on  WhichPCS=5
      settings: SourceProductName=NXP Model-Based Design Toolbox for MPC57xx MCUs
  Terminator : Terminator
  Terminator1 : Terminator
  Vector Concatenate1 : Concatenate
  wires:
  Vector Concatenate1/1 -> SPI_Master_Transfer_To1/1
  SPI_Master_Transfer_To1/1 -> Demux1/1
  Demux1/2 -> Data Type Conversion4/1
  Data Type Conversion3/1 -> Terminator/1
  Data Type Conversion4/1 -> Terminator1/1
  Demux1/1 -> Data Type Conversion3/1
  If Action Subsystem1/1(Out1) -> Vector Concatenate1/1
  If Action Subsystem1/2(Out2) -> Vector Concatenate1/2

== system ECU1119_18b_st/GPIO /SPI0: LS09_14_15_16_1_2_11_4/LS_CTRL1 ==
  Enable : EnablePort
  Data Type Conversion3 : DataTypeConversion
  Data Type Conversion4 : DataTypeConversion
  Demux1 : Demux  Outputs=2
  If Action Subsystem1 : Subsystem  TreatAsAtomicUnit=on
  SPI_Master_Transfer_To1 : mbd_mpc574x_ec_toolbox/Communication Blocks/SPI Blocks/SPI_Master_Transfer  Priority=2  InstanceNumber=0  xfermode=Non blocking  timeout=50  spi_upd=on  WhichPCS=1
      settings: SourceProductName=NXP Model-Based Design Toolbox for MPC57xx MCUs
  Terminator : Terminator
  Terminator1 : Terminator
  Vector Concatenate1 : Concatenate
  wires:
  Demux1/1 -> Data Type Conversion3/1
  Data Type Conversion4/1 -> Terminator1/1
  Data Type Conversion3/1 -> Terminator/1
  Demux1/2 -> Data Type Conversion4/1
  SPI_Master_Transfer_To1/1 -> Demux1/1
  Vector Concatenate1/1 -> SPI_Master_Transfer_To1/1
  If Action Subsystem1/2(Out2) -> Vector Concatenate1/2
  If Action Subsystem1/1(Out1) -> Vector Concatenate1/1

== system ECU1119_18b_st/GPIO /SPI3: LS03_06_07_08_10_12_13_17_18_19/Subsystem ==
  Enable : EnablePort
  Data Type Conversion : DataTypeConversion  OutDataTypeStr=uint8
  Data Type Conversion1 : DataTypeConversion  OutDataTypeStr=uint8
  Demux2 : Demux  Outputs=2
  SPI_Master_Transfer_To2 : mbd_mpc574x_ec_toolbox/Communication Blocks/SPI Blocks/SPI_Master_Transfer  Priority=2  InstanceNumber=3  xfermode=Non blocking  timeout=50  spi_upd=on  WhichPCS=3
      settings: SourceProductName=NXP Model-Based Design Toolbox for MPC57xx MCUs
  Terminator2 : Terminator
  Terminator3 : Terminator
  Vector Concatenate2 : Concatenate
  控制 : Subsystem  TreatAsAtomicUnit=on
  wires:
  Data Type Conversion1/1 -> Terminator3/1
  控制/2(Out2) -> Vector Concatenate2/2
  Demux2/1 -> Data Type Conversion/1
  Vector Concatenate2/1 -> SPI_Master_Transfer_To2/1
  Demux2/2 -> Data Type Conversion1/1
  Data Type Conversion/1 -> Terminator2/1
  控制/1(Out1) -> Vector Concatenate2/1
  SPI_Master_Transfer_To2/1 -> Demux2/1

== system ECU1119_18b_st/Initialization & SPI timer1/CS1 LS/Subsystem ==
  Data Store Read : DataStoreRead  DataStoreName=SPIO_CS1_InitFlg
  Merge : Merge  Inputs=3
  Merge1 : Merge  Inputs=3
  SPI_en : Subsystem  TreatAsAtomicUnit=on
  Switch Case : SwitchCase  CaseConditions={1,2,3}  ShowDefaultCase=off
  "clear " : Subsystem  TreatAsAtomicUnit=on
  confi_enbit : Subsystem  TreatAsAtomicUnit=on
  Out1 : Outport
  Out2 : Outport  Port=2
  wires:
  confi_enbit/1(Out1) -> Merge/3
  SPI_en/1(Out1) -> Merge/2
  "clear "/2(Out2) -> Merge1/1
  confi_enbit/2(Out2) -> Merge1/3
  "clear "/1(Out1) -> Merge/1
  Switch Case/1 -> "clear "/Action
  Switch Case/3 -> confi_enbit/Action
  Merge1/1 -> Out2/1
  Switch Case/2 -> SPI_en/Action
  SPI_en/2(Out2) -> Merge1/2
  Data Store Read/1 -> Switch Case/1
  Merge/1 -> Out1/1

== system ECU1119_18b_st/Initialization & SPI timer1/CS3 LS/Subsystem ==
  In1 : Inport
  In2 : Inport  Port=2
  A组配置 : Subsystem  TreatAsAtomicUnit=on
  B组配置 : Subsystem  TreatAsAtomicUnit=on
  Data Store Read : DataStoreRead  DataStoreName=SPI3_CTRL1
  Merge : Merge  Inputs=3
  Merge1 : Merge  Inputs=3
  Switch Case : SwitchCase  CaseConditions={1,2,3}  ShowDefaultCase=off
  Out1 : Outport
  Out2 : Outport  Port=2
  Out3 : Outport  Port=3
  wires:
  Switch Case/2 -> B组配置/Action
  Merge1/1 -> Out3/1
  A组配置/2(Out2) -> Merge1/1
  In2/1 -> Merge1/3
  Data Store Read/1 -> Switch Case/1
  B组配置/1(Out1) -> Merge/2
  Merge/1 -> Out2/1
  Switch Case/3 -> Out1/1
  A组配置/1(Out1) -> Merge/1
  B组配置/2(Out2) -> Merge1/2
  Switch Case/1 -> A组配置/Action
  In1/1 -> Merge/3

== system ECU1119_18b_st/Initialization & SPI timer1/CS5 LS/Subsystem ==
  Data Store Read : DataStoreRead  DataStoreName=SPIO_CS1_InitFlg
  Merge : Merge  Inputs=3
  Merge1 : Merge  Inputs=3
  SPI_en : Subsystem  TreatAsAtomicUnit=on
  Switch Case : SwitchCase  CaseConditions={1,2,3}  ShowDefaultCase=off
  "clear " : Subsystem  TreatAsAtomicUnit=on
  confi_enbit : Subsystem  TreatAsAtomicUnit=on
  Out1 : Outport
  Out2 : Outport  Port=2
  wires:
  confi_enbit/1(Out1) -> Merge/3
  SPI_en/1(Out1) -> Merge/2
  "clear "/2(Out2) -> Merge1/1
  confi_enbit/2(Out2) -> Merge1/3
  "clear "/1(Out1) -> Merge/1
  Switch Case/1 -> "clear "/Action
  Switch Case/3 -> confi_enbit/Action
  Merge1/1 -> Out2/1
  Switch Case/2 -> SPI_en/Action
  SPI_en/2(Out2) -> Merge1/2
  Data Store Read/1 -> Switch Case/1
  Merge/1 -> Out1/1

== system ECU1119_18b_st/SPI_EEPROM/SPI_write/SPI_enable ==
  Action Port : ActionPort
  Constant1 : Constant  Value=2
  Data Store Write : DataStoreWrite  DataStoreName=Write_Ctrl
  Data Type Conversion : DataTypeConversion  OutDataTypeStr=uint8
  Data Type Conversion3 : DataTypeConversion
  Data Type Conversion8 : DataTypeConversion
  Demux1 : Demux  Outputs=1
  SPI_Master_Transfer_To1 : mbd_mpc574x_ec_toolbox/Communication Blocks/SPI Blocks/SPI_Master_Transfer  Priority=2  InstanceNumber=0  xfermode=Non blocking  timeout=50  spi_upd=on  WhichPCS=0
      settings: SourceProductName=NXP Model-Based Design Toolbox for MPC57xx MCUs
  Terminator : Terminator
  Vector Concatenate1 : Concatenate  NumInputs=1
  write_enable : Constant  Value=6  OutDataTypeStr=uint8
  wires:
  Data Type Conversion3/1 -> Terminator/1  "r8"
  SPI_Master_Transfer_To1/1 -> Demux1/1
  Demux1/1 -> Data Type Conversion3/1
  Vector Concatenate1/1 -> SPI_Master_Transfer_To1/1
  write_enable/1 -> Data Type Conversion/1
  Data Type Conversion/1 -> Vector Concatenate1/1  "d8"
  Constant1/1 -> Data Type Conversion8/1
  Data Type Conversion8/1 -> Data Store Write/1

== system ECU1119_18b_st/SPI_EEPROM/SPI_write/SPI_write ==
  Action Port : ActionPort
  "Address_High " : Constant  Value=hex2dec('FF')  OutDataTypeStr=uint8
  Address_Low : Constant  Value=hex2dec('FF')
  Constant1 : Constant
  Data Store Read : DataStoreRead  DataStoreName=A_write
  Data Store Write : DataStoreWrite  DataStoreName=Write_Ctrl
  Data Type Conversion{,1..2,5} (4 alike) : DataTypeConversion  OutDataTypeStr=uint8
  Data Type Conversion{3..4,6..8} (5 alike) : DataTypeConversion
  Demux1 : Demux
  SPI_Master_Transfer_To1 : mbd_mpc574x_ec_toolbox/Communication Blocks/SPI Blocks/SPI_Master_Transfer  Priority=2  InstanceNumber=0  xfermode=Non blocking  timeout=50  spi_upd=on  WhichPCS=0
      settings: SourceProductName=NXP Model-Based Design Toolbox for MPC57xx MCUs
  Terminator{,1..3} (4 alike) : Terminator
  Vector Concatenate1 : Concatenate  NumInputs=4
  write_set : Constant  Value=2  OutDataTypeStr=uint8
  wires:
  Data Type Conversion4/1 -> Terminator1/1  "r5"
  Data Type Conversion3/1 -> Terminator/1  "r4"
  SPI_Master_Transfer_To1/1 -> Demux1/1
  Demux1/1 -> Data Type Conversion3/1
  Vector Concatenate1/1 -> SPI_Master_Transfer_To1/1
  Demux1/2 -> Data Type Conversion4/1
  Address_Low/1 -> Data Type Conversion5/1
  Data Type Conversion/1 -> Vector Concatenate1/1  "d4"
  Data Type Conversion1/1 -> Vector Concatenate1/2  "d5"
  write_set/1 -> Data Type Conversion/1
  "Address_High "/1 -> Data Type Conversion1/1
  Data Store Read/1 -> Data Type Conversion2/1
  Constant1/1 -> Data Type Conversion8/1
  Data Type Conversion5/1 -> Vector Concatenate1/3  "d6"
  Data Type Conversion2/1 -> Vector Concatenate1/4  "d7"
  Data Type Conversion6/1 -> Terminator2/1  "r6"
  Demux1/3 -> Data Type Conversion6/1
  Data Type Conversion7/1 -> Terminator3/1  "r7"
  Demux1/4 -> Data Type Conversion7/1
  Data Type Conversion8/1 -> Data Store Write/1

== system ECU1119_18b_st/SigIn/CAN2/Obj_Fast_Fb1 ==
  ID : Inport
  Data : Inport  Port=2
  length : Inport  Port=3
  timestamp : Inport  Port=4
  Switch Case : SwitchCase  CaseConditions={257}  ShowDefaultCase=off
  UNPACK : Subsystem  TreatAsAtomicUnit=on
  Message : Outport
  wires:
  UNPACK/1(Message) -> Message/1
  length/1 -> UNPACK/3(length)
  timestamp/1 -> UNPACK/4(timestamp)
  Data/1 -> UNPACK/2(data)
  ID/1 -> Switch Case/1, UNPACK/1(ID)
  Switch Case/1 -> UNPACK/Action

== system ECU1119_18b_st/SigIn/CAN2/Obj_Fast_Fb2 ==
  ID : Inport
  Data : Inport  Port=2
  length : Inport  Port=3
  timestamp : Inport  Port=4
  Switch Case : SwitchCase  CaseConditions={258}  ShowDefaultCase=off
  UNPACK : Subsystem  TreatAsAtomicUnit=on
  Message : Outport
  wires:
  Switch Case/1 -> UNPACK/Action
  ID/1 -> UNPACK/1(ID), Switch Case/1
  Data/1 -> UNPACK/2(data)
  timestamp/1 -> UNPACK/4(timestamp)
  length/1 -> UNPACK/3(length)
  UNPACK/1(Message) -> Message/1

== system ECU1119_18b_st/SigIn/CAN2/Obj_Slow_Fb1 ==
  ID : Inport
  Data : Inport  Port=2
  length : Inport  Port=3
  timestamp : Inport  Port=4
  Switch Case : SwitchCase  CaseConditions={261}  ShowDefaultCase=off
  UNPACK : Subsystem  TreatAsAtomicUnit=on
  Message : Outport
  wires:
  Switch Case/1 -> UNPACK/Action
  ID/1 -> UNPACK/1(ID), Switch Case/1
  Data/1 -> UNPACK/2(data)
  timestamp/1 -> UNPACK/4(timestamp)
  length/1 -> UNPACK/3(length)
  UNPACK/1(Message) -> Message/1

== system ECU1119_18b_st/SigIn/CAN2/Obj_Slow_Fb2 ==
  ID : Inport
  Data : Inport  Port=2
  length : Inport  Port=3
  timestamp : Inport  Port=4
  Switch Case : SwitchCase  CaseConditions={262}  ShowDefaultCase=off
  UNPACK : Subsystem  TreatAsAtomicUnit=on
  Message : Outport
  wires:
  UNPACK/1(Message) -> Message/1
  length/1 -> UNPACK/3(length)
  timestamp/1 -> UNPACK/4(timestamp)
  Data/1 -> UNPACK/2(data)
  ID/1 -> Switch Case/1, UNPACK/1(ID)
  Switch Case/1 -> UNPACK/Action

== system ECU1119_18b_st/SigIn/CAN2/Obj_Temp_Fb1 ==
  ID : Inport
  Data : Inport  Port=2
  length : Inport  Port=3
  timestamp : Inport  Port=4
  Switch Case : SwitchCase  CaseConditions={259}  ShowDefaultCase=off
  UNPACK : Subsystem  TreatAsAtomicUnit=on
  Message : Outport
  wires:
  UNPACK/1(Message) -> Message/1
  length/1 -> UNPACK/3(length)
  timestamp/1 -> UNPACK/4(timestamp)
  Data/1 -> UNPACK/2(data)
  ID/1 -> Switch Case/1, UNPACK/1(ID)
  Switch Case/1 -> UNPACK/Action

== system ECU1119_18b_st/SigIn/CAN2/Obj_Temp_Fb2 ==
  ID : Inport
  Data : Inport  Port=2
  length : Inport  Port=3
  timestamp : Inport  Port=4
  Switch Case : SwitchCase  CaseConditions={260}  ShowDefaultCase=off
  UNPACK : Subsystem  TreatAsAtomicUnit=on
  Message : Outport
  wires:
  Switch Case/1 -> UNPACK/Action
  ID/1 -> UNPACK/1(ID), Switch Case/1
  Data/1 -> UNPACK/2(data)
  timestamp/1 -> UNPACK/4(timestamp)
  length/1 -> UNPACK/3(length)
  UNPACK/1(Message) -> Message/1

== system ECU1119_18b_st/SigIn/DI/DI_31_32_33_34 ==
  note: DI PWM PULLUP
  note: DI PWM PULLDOWN
  DI31 : mbd_mpc574x_ec_toolbox/GPIO Blocks/Digital_Input  gpio_pin=PTF0: [SIUL2_GPIO80 | General Purpose IO PF[0]]  pull_resistor=None
      settings: SourceProductName=NXP Model-Based Design Toolbox for MPC57xx MCUs
  DI32 : mbd_mpc574x_ec_toolbox/GPIO Blocks/Digital_Input  gpio_pin=PTD1: [SIUL2_GPIO49 | General Purpose IO PD[1]]  pull_resistor=None
      settings: SourceProductName=NXP Model-Based Design Toolbox for MPC57xx MCUs
  DI33 : mbd_mpc574x_ec_toolbox/GPIO Blocks/Digital_Input  gpio_pin=PTD2: [SIUL2_GPIO50 | General Purpose IO PD[2]]  pull_resistor=None
      settings: SourceProductName=NXP Model-Based Design Toolbox for MPC57xx MCUs
  DI34 : mbd_mpc574x_ec_toolbox/GPIO Blocks/Digital_Input  gpio_pin=PTC13: [SIUL2_GPIO45 | General Purpose IO PC[13]]  pull_resistor=None
      settings: SourceProductName=NXP Model-Based Design Toolbox for MPC57xx MCUs
  Data Store Write14 : DataStoreWrite  DataStoreName=DI31
  Data Store Write15 : DataStoreWrite  DataStoreName=DI32
  Data Store Write16 : DataStoreWrite  DataStoreName=DI33
  Data Store Write17 : DataStoreWrite  DataStoreName=DI34
  wires:
  DI34/1 -> Data Store Write17/1
  DI33/1 -> Data Store Write16/1
  DI32/1 -> Data Store Write15/1
  DI31/1 -> Data Store Write14/1

== system ECU1119_18b_st/SigIn/PWM/PWM_PTS1 ==
  Add : Sum  Inputs=+-  AccumDataTypeStr=single
  Add1 : Sum  Inputs=+-  AccumDataTypeStr=single
  Data Store Memory : DataStoreMemory  DataStoreName=pts1_pwm_cnt  ReadBeforeWriteMsg=warning  WriteAfterWriteMsg=warning  WriteAfterReadMsg=warning  ShowAdditionalParam=off  OutDataTypeStr=uint8
  Data Store Memory2 : DataStoreMemory  DataStoreName=pts1_fifo_1_vect  ReadBeforeWriteMsg=warning  WriteAfterWriteMsg=warning  WriteAfterReadMsg=warning  InitialValue=[0 0 0 0 0 0 0 0]  ShowAdditionalParam=off  OutDataTypeStr=uint16
  Data Store Memory4 : DataStoreMemory  DataStoreName=pts1_fifo_0_vect  ReadBeforeWriteMsg=warning  WriteAfterWriteMsg=warning  WriteAfterReadMsg=warning  InitialValue=[0 0 0 0 0 0 0 0]  ShowAdditionalParam=off  OutDataTypeStr=uint16
  Data Store Read : DataStoreRead  DataStoreName=pts1_fifo_0_vect  DataStoreElements=pts1_fifo_0_vect(2)#pts1_fifo_0_vect(1)
  Data Store Read1 : DataStoreRead  DataStoreName=pts1_fifo_1_vect  DataStoreElements=pts1_fifo_1_vect(1)
  Data Store Read2 : DataStoreRead  DataStoreName=pts1_fifo_0_vect  DataStoreElements=pts1_fifo_0_vect(1)
  Data Store Write3 : DataStoreWrite  DataStoreName=pts1_fifo_0_vect
  Data Store Write5 : DataStoreWrite  DataStoreName=pts1_fifo_1_vect
  Divide : Product  Inputs=*/  OutDataTypeStr=single
  Divide1 : Product  Inputs=*//
  Freq_MC : Constant  Value=80000000  OutDataTypeStr=single
  Prescaler : Constant  Value=32  OutDataTypeStr=single
  Subsystem : Subsystem
  Subsystem_capture : Subsystem
  Terminator1 : Terminator
  Terminator2 : Terminator
  eTimer_ISR : mbd_mpc574x_ec_toolbox/Motor Control Blocks/eTIMER Blocks/eTimer_ISR_Handler  etimerModule=1  etimerInterrupt=Channel Interrupt  etimerChannel=2  etimerIsrPriority=14
      settings: SourceProductName=NXP Model-Based Design Toolbox for MPC57xx MCUs
  DC : Outport
  freq : Outport  Port=2
  wires:
  eTimer_ISR/2 -> Subsystem_capture/1(In1)
  Subsystem_capture/1(Out1) -> Terminator1/1
  Subsystem_capture/3(Out3) -> Terminator2/1
  Subsystem_capture/4(Out4) -> Data Store Write5/1
  Subsystem_capture/2(Out2) -> Data Store Write3/1
  eTimer_ISR/1 -> Subsystem_capture/Trigger
  Prescaler/1 -> Divide1/2
  Add/1 -> Divide/2, Divide1/3
  Data Store Read1/1 -> Add1/1
  Data Store Read/2 -> Add/2
  Freq_MC/1 -> Divide1/1
  Add1/1 -> Divide/1
  Data Store Read2/1 -> Add1/2
  Divide1/1 -> freq/1
  Data Store Read/1 -> Add/1
  Divide/1 -> Subsystem/1(In1)
  Subsystem/1(Out1) -> DC/1
